simulink library "conventional_airplane_aerodynamics_lib"  (R2018b)
settings: Solver=VariableStepAuto  StartTime=0.0  StopTime=10.0  RelTol=1e-3
undefined symbols (not defined in the file or in its folder): aero
libraries: simple_wing_lib x3, flight_parameters_lib x2, simpleFuselage_lib x1
settings Model: Creator=Ybeyer  LastModifiedBy=yannic
settings SFSimCC: SimUseLocalCustomCode=off
settings RTWCC: RTWUseLocalCustomCode=off
settings CodeAppCC: StateflowObjectComments=on

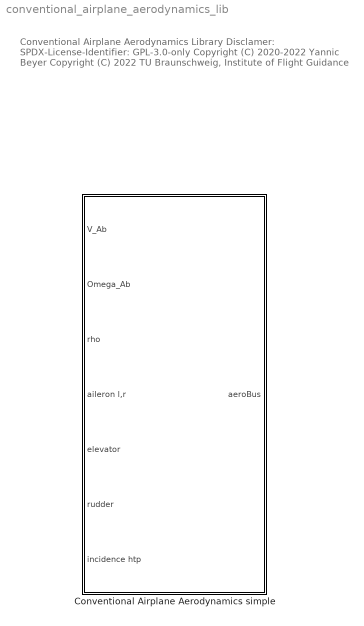
== system conventional_airplane_aerodynamics_lib ==
  note: Conventional Airplane Aerodynamics Library
      |
      | Disclamer:
      | SPDX-License-Identifier: GPL-3.0-only
      |
      | Copyright (C) 2020-2022 Yannic Beyer
      | Copyright (C) 2022 TU Braunschweig, Institute of Flight Guidance
  Conventional Airplane Aerodynamics simple : Subsystem  mask{aeroStruct=aero, xyz_cg_c=zeros(3,1)}
      mask prompts: aeroStruct "aerodynamics struct of the conventional airplane"; xyz_cg_c "center of gravity position in c frame, m"
      mask DialogControl DescGroupVar Prompt: Conventional Airplane Aerodynamics simple
      mask DialogControl DescTextVar Prompt: Contains three 2 point wing models for the main wing, the horizontal tailplane and the vertical tailplane. See conventionalAirplaneLoadParams for information about the struct.

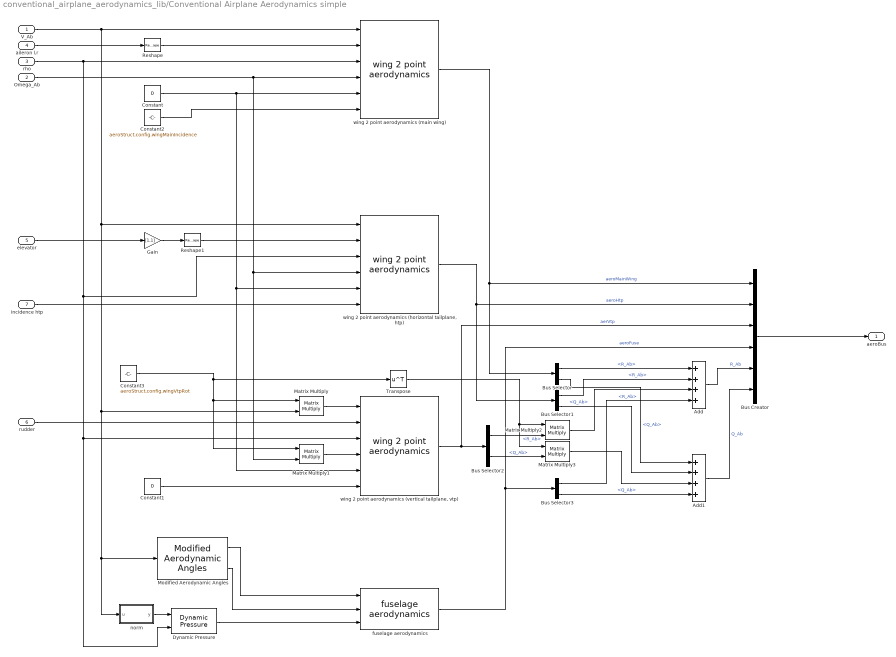
== system conventional_airplane_aerodynamics_lib/Conventional Airplane Aerodynamics simple ==
  V_Ab : Inport
  Omega_Ab : Inport  Port=2
  rho : Inport  Port=3
  aileron l,r : Inport  Port=4
  elevator : Inport  Port=5
  rudder : Inport  Port=6
  incidence htp : Inport  Port=7
  Add : Sum  Inputs=++++
  Add1 : Sum  Inputs=++++
  Bus Creator : BusCreator  Inputs=6
  Bus Selector : BusSelector  OutputSignals=dynamicsBody.R_Ab,dynamicsBody.Q_Ab
  Bus Selector1 : BusSelector  OutputSignals=dynamicsBody.R_Ab,dynamicsBody.Q_Ab
  Bus Selector2 : BusSelector  OutputSignals=dynamicsBody.R_Ab,dynamicsBody.Q_Ab
  Bus Selector3 : BusSelector  OutputSignals=R_Ab,Q_Ab
  Constant : Constant  Value=0
  Constant1 : Constant  Value=0
  Constant2 : Constant  Value=aeroStruct.config.wingMainIncidence
  Constant3 : Constant  Value=aeroStruct.config.wingVtpRot
  Dynamic Pressure : flight_parameters_lib/Dynamic Pressure
      settings: SourceProductName=LADAC
  Gain : Gain  Gain=[1,1]
  Matrix Multiply{,1..3} (4 alike) : Product  Multiplication=Matrix(*)
  Modified Aerodynamic Angles : flight_parameters_lib/Modified Aerodynamic Angles  SystemSampleTime=-1
      settings: SourceProductName=LADAC
  Reshape : Reshape  OutputDimensionality=Row vector (2-D)
  Reshape1 : Reshape  OutputDimensionality=Row vector (2-D)
  Transpose : Math  Operator=transpose  SaturateOnIntegerOverflow=on
  fuselage aerodynamics : simpleFuselage_lib/fuselage aerodynamics  simple_fuselage=aeroStruct.fuse
      settings: SourceProductName=LADAC
  norm : MATLAB Function  TreatAsAtomicUnit=on
  "wing 2 point aerodynamics (horizontal tailplane, htp)" : simple_wing_lib/wing 2 point aerodynamics  wingStruct=aeroStruct.wingHtp  xyz_wing_c=aeroStruct.config.wingHtpPos  xyz_cg_c=xyz_cg_c
      settings: SourceProductName=LADAC
  wing 2 point aerodynamics (main wing) : simple_wing_lib/wing 2 point aerodynamics  wingStruct=aeroStruct.wingMain  xyz_wing_c=aeroStruct.config.wingMainPos  xyz_cg_c=xyz_cg_c
      settings: SourceProductName=LADAC
  "wing 2 point aerodynamics (vertical tailplane, vtp)" : simple_wing_lib/wing 2 point aerodynamics  wingStruct=aeroStruct.wingVtp  xyz_wing_c=aeroStruct.config.wingVtpPos  xyz_cg_c=xyz_cg_c
      settings: SourceProductName=LADAC
  aeroBus : Outport
  wires:
  V_Ab/1 -> Matrix Multiply/2, norm/1(u), Modified Aerodynamic Angles/1, "wing 2 point aerodynamics (horizontal tailplane, htp)"/1, wing 2 point aerodynamics (main wing)/1
  aileron l,r/1 -> Reshape/1
  rho/1 -> wing 2 point aerodynamics (main wing)/3, "wing 2 point aerodynamics (horizontal tailplane, htp)"/3, Dynamic Pressure/2, "wing 2 point aerodynamics (vertical tailplane, vtp)"/3
  Dynamic Pressure/1 -> fuselage aerodynamics/3
  Constant/1 -> wing 2 point aerodynamics (main wing)/5, "wing 2 point aerodynamics (vertical tailplane, vtp)"/5, "wing 2 point aerodynamics (horizontal tailplane, htp)"/5
  Constant2/1 -> wing 2 point aerodynamics (main wing)/6
  incidence htp/1 -> "wing 2 point aerodynamics (horizontal tailplane, htp)"/6
  Constant1/1 -> "wing 2 point aerodynamics (vertical tailplane, vtp)"/6
  Modified Aerodynamic Angles/1 -> fuselage aerodynamics/1
  Modified Aerodynamic Angles/2 -> fuselage aerodynamics/2
  norm/1(y) -> Dynamic Pressure/1
  elevator/1 -> Gain/1
  Gain/1 -> Reshape1/1
  rudder/1 -> "wing 2 point aerodynamics (vertical tailplane, vtp)"/2
  wing 2 point aerodynamics (main wing)/1 -> Bus Selector/1, Bus Creator/1  "aeroMainWing"
  "wing 2 point aerodynamics (horizontal tailplane, htp)"/1 -> Bus Creator/2, Bus Selector1/1  "aeroHtp"
  "wing 2 point aerodynamics (vertical tailplane, vtp)"/1 -> Bus Creator/3, Bus Selector2/1  "aerVtp"
  Bus Creator/1 -> aeroBus/1
  fuselage aerodynamics/1 -> Bus Creator/4, Bus Selector3/1  "aeroFuse"
  Reshape/1 -> wing 2 point aerodynamics (main wing)/2
  Reshape1/1 -> "wing 2 point aerodynamics (horizontal tailplane, htp)"/2
  Matrix Multiply/1 -> "wing 2 point aerodynamics (vertical tailplane, vtp)"/1
  Constant3/1 -> Matrix Multiply1/1, Matrix Multiply/1, Transpose/1
  Matrix Multiply1/1 -> "wing 2 point aerodynamics (vertical tailplane, vtp)"/4
  Omega_Ab/1 -> wing 2 point aerodynamics (main wing)/4, Matrix Multiply1/2, "wing 2 point aerodynamics (horizontal tailplane, htp)"/4
  Bus Selector/1 -> Add/1  "<R_Ab>"
  Bus Selector1/1 -> Add/2  "<R_Ab>"
  Matrix Multiply2/1 -> Add/3
  Bus Selector3/1 -> Add/4  "<R_Ab>"
  Bus Selector3/2 -> Add1/4  "<Q_Ab>"
  Matrix Multiply3/1 -> Add1/3
  Bus Selector1/2 -> Add1/2  "<Q_Ab>"
  Bus Selector/2 -> Add1/1  "<Q_Ab>"
  Add/1 -> Bus Creator/5  "R_Ab"
  Add1/1 -> Bus Creator/6  "Q_Ab"
  Bus Selector2/1 -> Matrix Multiply2/2  "<R_Ab>"
  Bus Selector2/2 -> Matrix Multiply3/2  "<Q_Ab>"
  Transpose/1 -> Matrix Multiply3/1, Matrix Multiply2/1

== matlab function conventional_airplane_aerodynamics_lib/Conventional Airplane Aerodynamics simple/norm ==
  data: u input; y output
function y = fcn(u)
y = norm(u,2);
